simulink model "Gr2_Ex7_2LinkRobot_TaskSpacePD"  (R2024b)
settings: Solver=VariableStepAuto  StartTime=0.0  StopTime=5  RelTol=1e-3
values from neighbouring files (symbols this model uses):
  dq0 = [0; 0]    [Gr2_Ex4_5_6_main.m]    (also in Gr2_Ex7_main.m; Gr2_Ex8_main.m)
  ellipse = [0.15 0.2 0.15 0.1 1/3]    [Gr2_Ex7_main.m]
  Kd = 10    [Gr2_Ex7_main.m]    (also in Gr2_Ex8_main.m)
  Kp = 100    [Gr2_Ex7_main.m]    (also in Gr2_Ex8_main.m; Gr3_Ex1_main.m = 10; Gr3_Ex2_main.m = 10)
  modelParameters = [m1, m2, l1, l2, g0, Fv]    [Gr2_Ex4_5_6_main.m]    (also in Gr2_Ex7_main.m = [m1 m2 l1 l2 g0 Fv]; Gr2_Ex8_main.m = [m1 m2 l1 l2 g0 Fv])
  q0 = [pi/2; pi/4]    [Gr2_Ex4_5_6_main.m]    (also in Gr2_Ex7_main.m = [0; pi/2]; Gr2_Ex8_main.m = [q1; q2])
  tau_e = [0, 0]    [Gr2_Ex4_5_6_main.m]    (also in Gr2_Ex7_main.m = [0; 0]; Gr2_Ex8_main.m = [0; 0])
settings Model: Creator=UX434  LastModifiedBy=UX434

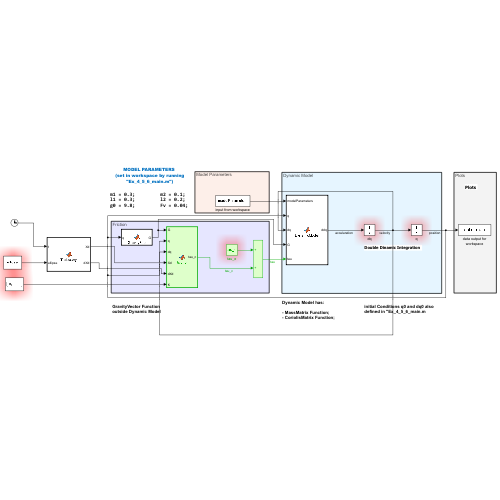
[thumbnail: Simulink's stored preview of the top-level diagram]
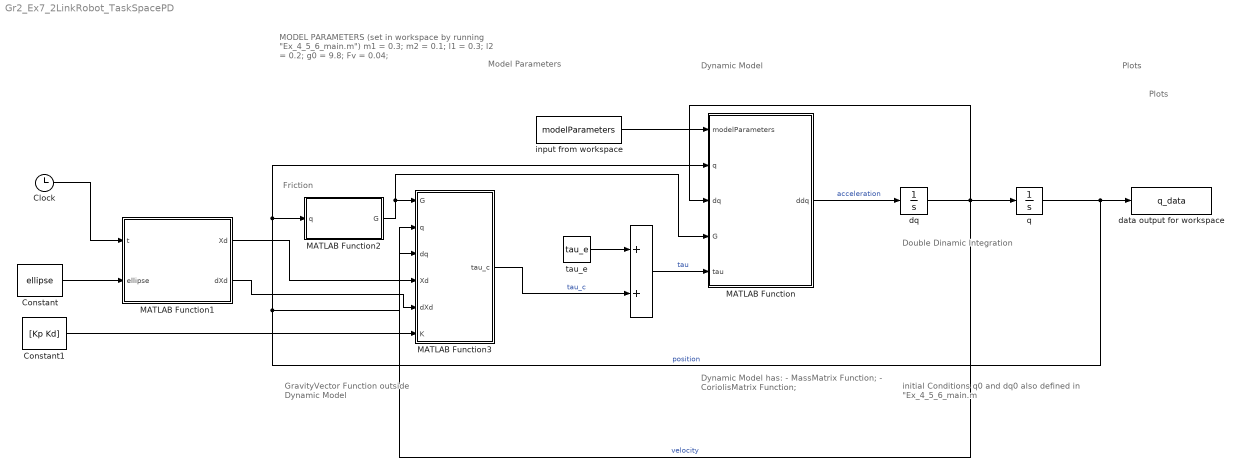
== system Gr2_Ex7_2LinkRobot_TaskSpacePD ==
  note: Plots
  note: Dynamic Model
  note: Friction
  note: Double Dinamic Integration
  note: Plots
  note: Dynamic Model has:
      |
      | - MassMatrix Function;
      | - CoriolisMatrix Function;
  note: GravityVector Function outside Dynamic Model
  note: Model Parameters
  note: MODEL PARAMETERS
      | (set in workspace by running "Ex_4_5_6_main.m")
      |
      | m1 = 0.3; m2 = 0.1;
      | l1 = 0.3; l2 = 0.2;
      | g0 = 9.8; Fv = 0.04;
  note: initial Conditions q0 and dq0 also defined in "Ex_4_5_6_main.m
  " " : Sum
  Clock : Clock
  Constant : Constant  Value=ellipse  VectorParams1D=off
  Constant1 : Constant  Value=[Kp Kd]  VectorParams1D=off
  MATLAB Function : MATLAB Function  TreatAsAtomicUnit=on
  MATLAB Function1 : MATLAB Function  TreatAsAtomicUnit=on
  MATLAB Function2 : MATLAB Function  TreatAsAtomicUnit=on
  MATLAB Function3 : MATLAB Function  TreatAsAtomicUnit=on
  data output for workspace : ToWorkspace  VariableName=q_data  SampleTime=-1
      settings: Save2DSignal=2-D array (concatenate along first dimension)
  dq : Integrator  InitialCondition=dq0
  input from workspace : Constant  Value=modelParameters
  q : Integrator  InitialCondition=q0
  tau_e : Constant  Value=tau_e
  wires:
  MATLAB Function/1(ddq) -> dq/1  "acceleration"
  dq/1 -> q/1, MATLAB Function3/3(dq), MATLAB Function/3(dq)  "velocity"
  q/1 -> data output for workspace/1, MATLAB Function/2(q), MATLAB Function2/1(q), MATLAB Function3/2(q)  "position"
  MATLAB Function3/1(tau_c) -> " "/2  "tau_c"
  " "/1 -> MATLAB Function/5(tau)  "tau"
  tau_e/1 -> " "/1
  MATLAB Function2/1(G) -> MATLAB Function/4(G), MATLAB Function3/1(G)
  input from workspace/1 -> MATLAB Function/1(modelParameters)
  Constant/1 -> MATLAB Function1/2(ellipse)
  Clock/1 -> MATLAB Function1/1(t)
  Constant1/1 -> MATLAB Function3/6(K)
  MATLAB Function1/1(Xd) -> MATLAB Function3/4(Xd)
  MATLAB Function1/2(dXd) -> MATLAB Function3/5(dXd)

== matlab function Gr2_Ex7_2LinkRobot_TaskSpacePD/MATLAB Function1 ==
  data: t input; Xd output; ellipse input; dXd output
function [Xd, dXd] = Trajectory(t, ellipse)
    xc = ellipse(1);  yc = ellipse(2);
    mx = ellipse(3);  my = ellipse(4);
    w  = 2*pi*ellipse(5);
    Xd  = [xc + mx*cos(w*t);  yc + my*sin(w*t)];
    dXd = [-mx*w*sin(w*t);    my*w*cos(w*t)];

== matlab function Gr2_Ex7_2LinkRobot_TaskSpacePD/MATLAB Function ==
  data: modelParameters input; ddq output; q input; dq input; G input; tau input
function ddq= DynamicModel(modelParameters, q, dq, G, tau)

m1 = modelParameters(1);         m2 = modelParameters(2); 
l1 = modelParameters(3);         l2 = modelParameters(4); 
g0 = modelParameters(5);         Fv = modelParameters(6);

lc1 = l1/2;  lc2 = l2/2;
I1czz = m1*l1^2/12;  I2czz = m2*l2^2/12;

M = Gr2_Ex3_MassMatrix(q, m1, m2, l1, lc1, lc2, I1czz, I2czz);
C = Gr2_Ex3_CoriolisMatrix(q, dq, m2, l1, lc2);

ddq = M \ (tau - C*dq - G - Fv*dq);

== matlab function Gr2_Ex7_2LinkRobot_TaskSpacePD/MATLAB Function2 ==
  data: q input; G output
function G = GravityFnc(q)
m1 = 0.3;         m2 = 0.1; 
l1 = 0.3;         l2 = 0.2; 
g0 = 9.8;

lc1 = l1/2;  lc2 = l2/2; 

G = Gr2_Ex3_GravityVector(q, m1, m2, lc1, l1, lc2, g0);

== matlab function Gr2_Ex7_2LinkRobot_TaskSpacePD/MATLAB Function3 ==
  data: G input; q input; tau_c output; dq input; Xd input; dXd input; K input
function tau_c = tau_c(G, q, dq, Xd, dXd, K)
l1 = 0.3;  l2 = 0.2;
lc1 = l1/2;  lc2 = l2/2;
Kp = K(1);  Kd = K(2);

Jv = Gr2_Ex2_Jacobians(q, l1, l2, lc1, lc2);
Jv = Jv(1:2,:);                          % only x and y rows

X  = [l1*cos(q(1)) + l2*cos(q(1)+q(2));
      l1*sin(q(1)) + l2*sin(q(1)+q(2))];   % end-effector position
dX = Jv*dq;                               % end-effector velocity

F = Kp*(Xd - X) + Kd*(dXd - dX);          % task space PD (Kd = 0 -> P)
tau_c = G + Jv'*F;
